simulink model "mrca"  (R2026a)
settings: Solver=FixedStepDiscrete  FixedStep=0.0002
undefined symbols (not defined in the file): DiscIntNeverNeededParam
libraries: discretizing x1
settings Model: SILPILModeSetting=veronly  Creator=HomePC  LastModifiedBy=HomePC
settings RTWCC: SystemTargetFile=ert.tlc  TemplateMakefile=RTW.MSVCBuild  Toolchain=ESP32  BuildConfiguration=Faster Runs  Description=Create Visual C/C++ Solution File for Embedded Coder
settings ERTTargetCC: DynamicArrayContainerType=coder::array  GenerateSampleERTMain=on  SupportComplex=off

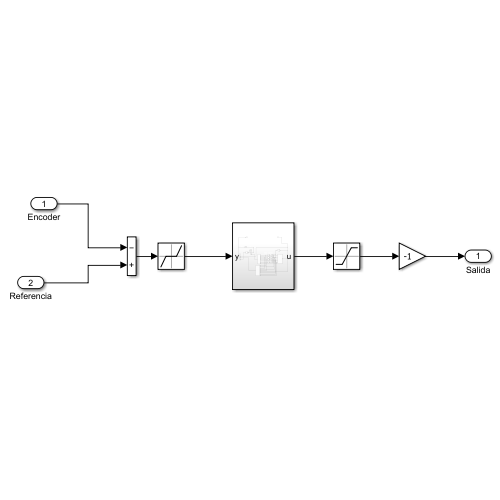
[thumbnail: Simulink's stored preview of the top-level diagram]
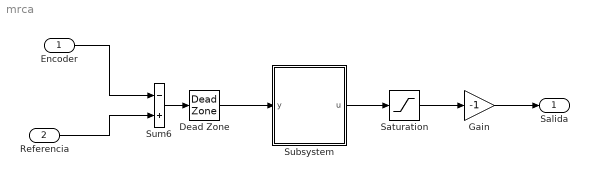
== system mrca ==
  Encoder : Inport
  Referencia : Inport  Port=2
  Dead Zone : DeadZone  LowerValue=-1  UpperValue=1
  Gain : Gain  Gain=-1
  Saturation : Saturate  UpperLimit=4095  LowerLimit=-4095  OutMin=[-4095]  OutMax=[4095]
  Subsystem : Subsystem
  Sum6 : Sum  Inputs=-+
  Salida : Outport
  wires:
  Referencia/1 -> Sum6/2
  Encoder/1 -> Sum6/1
  Sum6/1 -> Dead Zone/1
  Subsystem/1(u) -> Saturation/1
  Saturation/1 -> Gain/1
  Gain/1 -> Salida/1
  Dead Zone/1 -> Subsystem/1(y)

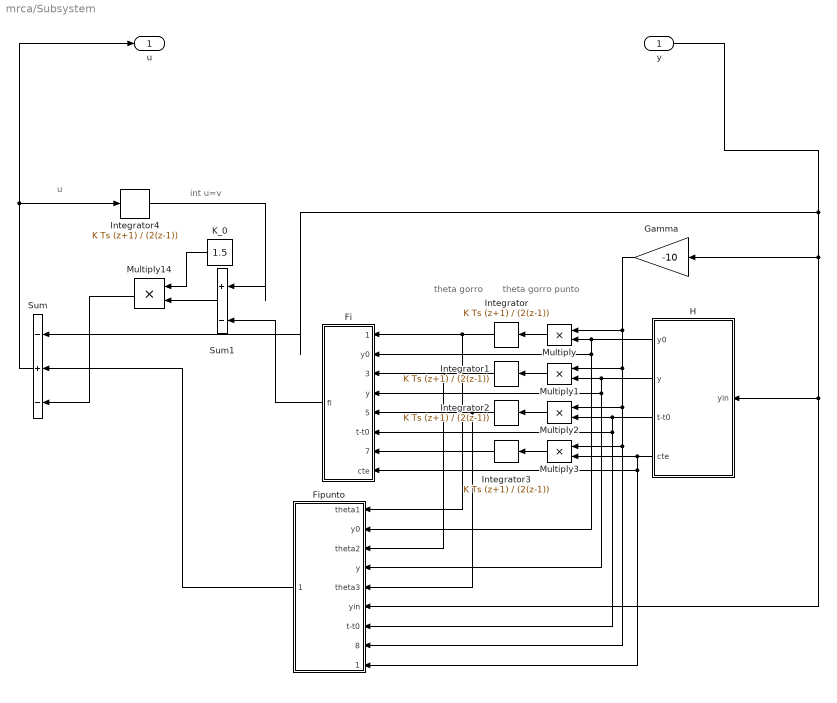
== system mrca/Subsystem ==
  note: int u=v
  note: u
  note: theta gorro
  note: theta gorro punto
  y : Inport
  Fi : Subsystem
  Fipunto : Subsystem
  Gamma : Gain  Gain=-10
  H : Subsystem
  Integrator : DiscreteIntegrator  IntegratorMethod=Integration: Trapezoidal  SampleTime=0.001  ICPrevOutput=DiscIntNeverNeededParam  ICPrevScaledInput=DiscIntNeverNeededParam  mask(DiscretizedDiscreteIntegrator){}
      mask init:
      | %tustin
  Integrator1 : DiscreteIntegrator  IntegratorMethod=Integration: Trapezoidal  SampleTime=0.001  ICPrevOutput=DiscIntNeverNeededParam  ICPrevScaledInput=DiscIntNeverNeededParam  mask(DiscretizedDiscreteIntegrator){}
      mask init:
      | %tustin
  Integrator2 : DiscreteIntegrator  IntegratorMethod=Integration: Trapezoidal  SampleTime=0.001  ICPrevOutput=DiscIntNeverNeededParam  ICPrevScaledInput=DiscIntNeverNeededParam  mask(DiscretizedDiscreteIntegrator){}
      mask init:
      | %tustin
  Integrator3 : DiscreteIntegrator  IntegratorMethod=Integration: Trapezoidal  SampleTime=0.001  ICPrevOutput=DiscIntNeverNeededParam  ICPrevScaledInput=DiscIntNeverNeededParam  mask(DiscretizedDiscreteIntegrator){}
      mask init:
      | %tustin
  Integrator4 : DiscreteIntegrator  IntegratorMethod=Integration: Trapezoidal  SampleTime=0.001  ICPrevOutput=DiscIntNeverNeededParam  ICPrevScaledInput=DiscIntNeverNeededParam  mask(DiscretizedDiscreteIntegrator){}
      mask init:
      | %tustin
  K_0 : Constant  Value=1.5  VectorParams1D=off  SampleTime=-1
  Multiply{,1..3,14} (5 alike) : Product
  Sum : Sum  Inputs=|-+-
  Sum1 : Sum  Inputs=|+-
  u : Outport  VectorParamsAs1DForOutWhenUnconnected=off
  wires:
  Fi/1(fi) -> Sum1/2
  y/1 -> Sum/1, Gamma/1, Fipunto/6(yin), H/1(yin)
  H/2(y) -> Fi/4(y), Fipunto/4(y), Multiply1/2
  Integrator3/1 -> Fi/7(theta4)
  Gamma/1 -> Multiply/1, Multiply1/1, Multiply2/1, Multiply3/1, Fipunto/8(-delta y)
  Multiply2/1 -> Integrator2/1
  Integrator2/1 -> Fipunto/5(theta3), Fi/5(theta3)
  H/1(y0) -> Fi/2(y0), Fipunto/2(y0), Multiply/2
  H/4(cte) -> Fipunto/9(1), Fi/8(cte), Multiply3/2
  Multiply1/1 -> Integrator1/1
  Multiply/1 -> Integrator/1
  K_0/1 -> Multiply14/1
  Multiply3/1 -> Integrator3/1
  H/3(t-t0) -> Fipunto/7(t-t0), Fi/6(t-t0), Multiply2/2
  Integrator4/1 -> Sum1/1
  Sum/1 -> u/1, Integrator4/1
  Integrator/1 -> Fipunto/1(theta1), Fi/1(theta1)
  Integrator1/1 -> Fi/3(theta2), Fipunto/3(theta2)
  Multiply14/1 -> Sum/3
  Fipunto/1(fi punto) -> Sum/2
  Sum1/1 -> Multiply14/2

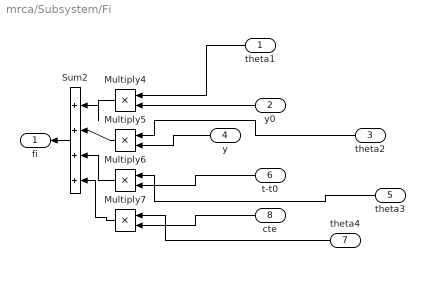
== system mrca/Subsystem/Fi ==
  theta1 : Inport
  y0 : Inport  Port=2
  theta2 : Inport  Port=3
  y : Inport  Port=4
  theta3 : Inport  Port=5
  t-t0 : Inport  Port=6
  theta4 : Inport  Port=7
  cte : Inport  Port=8
  Multiply{4..7} (4 alike) : Product
  Sum2 : Sum  Inputs=|++++
  fi : Outport  VectorParamsAs1DForOutWhenUnconnected=off
  wires:
  Multiply5/1 -> Sum2/2
  Multiply6/1 -> Sum2/3
  Multiply4/1 -> Sum2/1
  Sum2/1 -> fi/1
  Multiply7/1 -> Sum2/4
  theta1/1 -> Multiply4/1
  y0/1 -> Multiply4/2
  y/1 -> Multiply5/2
  theta2/1 -> Multiply5/1
  t-t0/1 -> Multiply6/2
  theta3/1 -> Multiply6/1
  cte/1 -> Multiply7/2
  theta4/1 -> Multiply7/1

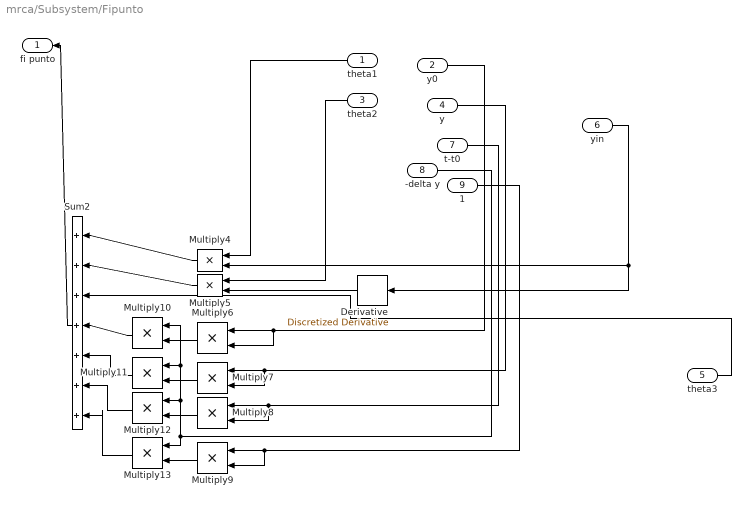
== system mrca/Subsystem/Fipunto ==
  theta1 : Inport
  y0 : Inport  Port=2
  theta2 : Inport  Port=3
  y : Inport  Port=4
  theta3 : Inport  Port=5
  yin : Inport  Port=6
  t-t0 : Inport  Port=7
  -delta y : Inport  Port=8
  1 : Inport  Port=9
  Derivative : discretizing/Discretized Derivative  method=tustin  SampleTime=0.001  Wc=1
  Multiply{4..13} (10 alike) : Product
  Sum2 : Sum  Inputs=|+++++++
  fi punto : Outport  VectorParamsAs1DForOutWhenUnconnected=off
  wires:
  Multiply11/1 -> Sum2/5
  yin/1 -> Derivative/1, Multiply4/2
  Multiply4/1 -> Sum2/1
  -delta y/1 -> Multiply10/1, Multiply11/1, Multiply12/1, Multiply13/1
  y/1 -> Multiply7/2, Multiply7/1
  Multiply9/1 -> Multiply13/2
  Multiply13/1 -> Sum2/7
  Multiply5/1 -> Sum2/2
  Multiply8/1 -> Multiply12/2
  t-t0/1 -> Multiply8/2, Multiply8/1
  1/1 -> Multiply9/2, Multiply9/1
  Multiply7/1 -> Multiply11/2
  Multiply10/1 -> Sum2/4
  Multiply6/1 -> Multiply10/2
  y0/1 -> Multiply6/2, Multiply6/1
  Sum2/1 -> fi punto/1
  Multiply12/1 -> Sum2/6
  theta1/1 -> Multiply4/1
  theta2/1 -> Multiply5/1
  Derivative/1 -> Multiply5/2
  theta3/1 -> Sum2/3

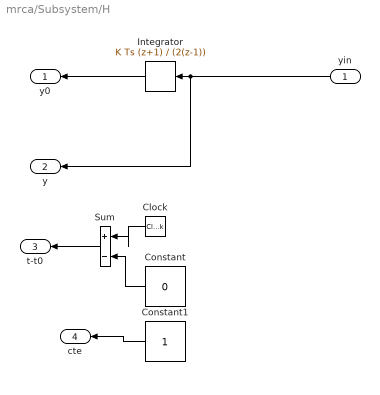
== system mrca/Subsystem/H ==
  yin : Inport
  Clock : DigitalClock  SampleTime=0.001
  Constant : Constant  Value=0  VectorParams1D=off  SampleTime=-1
  Constant1 : Constant  VectorParams1D=off  SampleTime=-1
  Integrator : DiscreteIntegrator  IntegratorMethod=Integration: Trapezoidal  SampleTime=0.001  ICPrevOutput=DiscIntNeverNeededParam  ICPrevScaledInput=DiscIntNeverNeededParam  mask(DiscretizedDiscreteIntegrator){}
      mask init:
      | %tustin
  Sum : Sum  Inputs=|+-
  y0 : Outport  VectorParamsAs1DForOutWhenUnconnected=off
  y : Outport  Port=2  VectorParamsAs1DForOutWhenUnconnected=off
  t-t0 : Outport  Port=3  VectorParamsAs1DForOutWhenUnconnected=off
  cte : Outport  Port=4  VectorParamsAs1DForOutWhenUnconnected=off
  wires:
  Clock/1 -> Sum/1
  Constant/1 -> Sum/2
  yin/1 -> y/1, Integrator/1
  Sum/1 -> t-t0/1
  Constant1/1 -> cte/1
  Integrator/1 -> y0/1
